simulink model "speed_ctrl"  (R2026a)
settings: Solver=ode4  StopTime=5  FixedStep=P_Ts/10
undefined symbols (not defined in the file or in its folder): P_alpha, P_cal, P_Dmax, P_dz, P_fm, P_Kb, P_Ki, P_Kp, P_omega_max, P_Rdn, P_Rup, P_Ts, PL_dz, PL_K, PL_Nrev, PL_tau, PL_td
settings Model: Creator=church  LastModifiedBy=church
settings DebuggingCC: ParameterPrecisionLossMsg=none

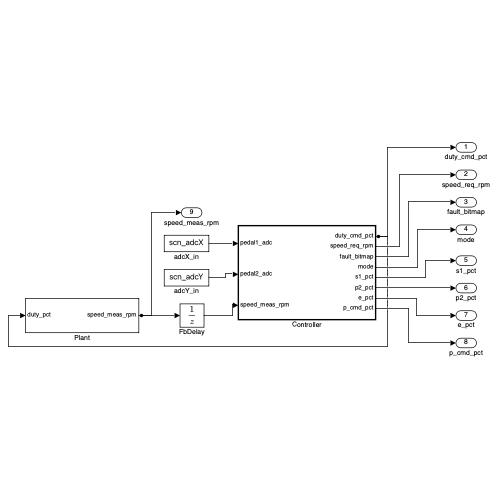
[thumbnail: Simulink's stored preview of the top-level diagram]
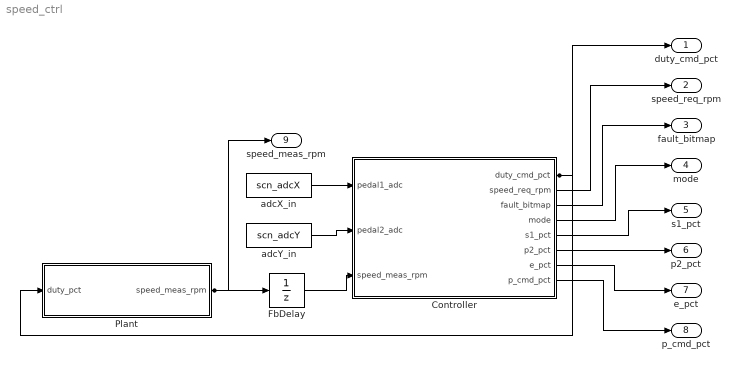
== system speed_ctrl ==
  Controller : Subsystem  TreatAsAtomicUnit=on
  FbDelay : UnitDelay  SampleTime=P_Ts
  Plant : Subsystem
  adcX_in : FromWorkspace  VariableName=scn_adcX  SampleTime=P_Ts  Interpolate=off  OutputAfterFinalValue=Holding final value
  adcY_in : FromWorkspace  VariableName=scn_adcY  SampleTime=P_Ts  Interpolate=off  OutputAfterFinalValue=Holding final value
  duty_cmd_pct : Outport  SampleTime=P_Ts
  speed_req_rpm : Outport  Port=2  SampleTime=P_Ts
  fault_bitmap : Outport  Port=3  SampleTime=P_Ts
  mode : Outport  Port=4  SampleTime=P_Ts
  s1_pct : Outport  Port=5  SampleTime=P_Ts
  p2_pct : Outport  Port=6  SampleTime=P_Ts
  e_pct : Outport  Port=7  SampleTime=P_Ts
  p_cmd_pct : Outport  Port=8  SampleTime=P_Ts
  speed_meas_rpm : Outport  Port=9  SampleTime=P_Ts
  wires:
  Controller/3(fault_bitmap) -> fault_bitmap/1
  Controller/5(s1_pct) -> s1_pct/1
  Controller/4(mode) -> mode/1
  Controller/6(p2_pct) -> p2_pct/1
  Controller/2(speed_req_rpm) -> speed_req_rpm/1
  Controller/7(e_pct) -> e_pct/1
  adcX_in/1 -> Controller/1(pedal1_adc)
  FbDelay/1 -> Controller/3(speed_meas_rpm)
  Plant/1(speed_meas_rpm) -> speed_meas_rpm/1, FbDelay/1
  Controller/8(p_cmd_pct) -> p_cmd_pct/1
  Controller/1(duty_cmd_pct) -> duty_cmd_pct/1, Plant/1(duty_pct)
  adcY_in/1 -> Controller/2(pedal2_adc)

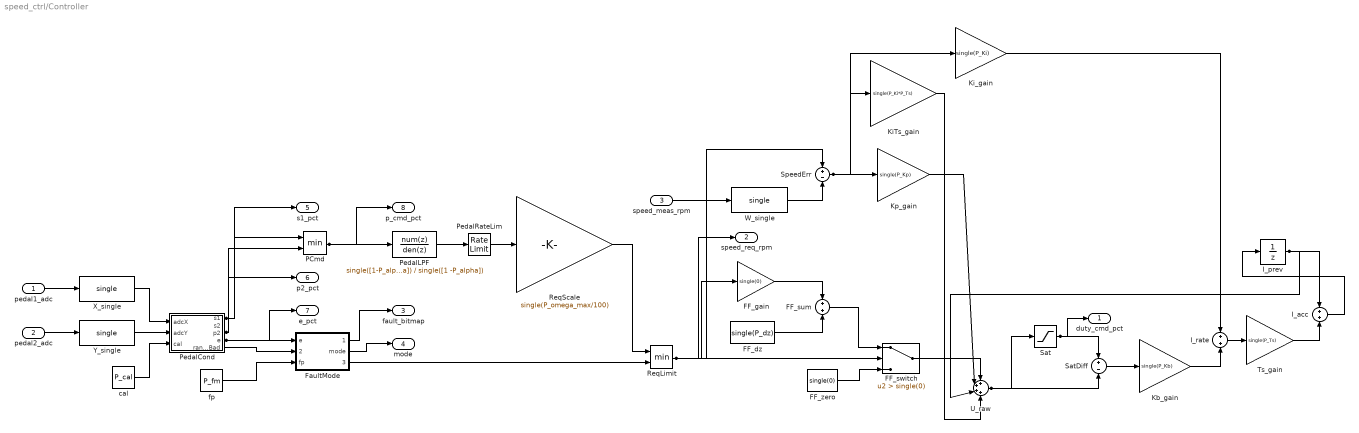
== system speed_ctrl/Controller ==
  pedal1_adc : Inport
  pedal2_adc : Inport  Port=2
  speed_meas_rpm : Inport  Port=3
  FF_dz : Constant  Value=single(P_dz)  OutDataTypeStr=single
  FF_gain : Gain  Gain=single(0)  ParamDataTypeStr=single
  FF_sum : Sum
  FF_switch : Switch  Criteria=u2 > Threshold  Threshold=single(0)  SaturateOnIntegerOverflow=off  InputSameDT=off
  FF_zero : Constant  Value=single(0)  OutDataTypeStr=single
  FaultMode : MATLAB Function  TreatAsAtomicUnit=on
  I_acc : Sum
  I_prev : UnitDelay  InitialCondition=single(0)  SampleTime=P_Ts
  I_rate : Sum
  Kb_gain : Gain  Gain=single(P_Kb)  ParamDataTypeStr=single
  KiTs_gain : Gain  Gain=single(P_Ki*P_Ts)  ParamDataTypeStr=single
  Ki_gain : Gain  Gain=single(P_Ki)  ParamDataTypeStr=single
  Kp_gain : Gain  Gain=single(P_Kp)  ParamDataTypeStr=single
  PCmd : MinMax  Inputs=2
  PedalCond : MATLAB Function  TreatAsAtomicUnit=on
  PedalLPF : DiscreteFilter  Numerator=single([1-P_alpha])  Denominator=single([1 -P_alpha])  SampleTime=P_Ts
  PedalRateLim : RateLimiter  RisingSlewLimit=single(P_Rup)  FallingSlewLimit=single(-P_Rdn)  SampleTimeMode=inherited
  ReqLimit : MinMax  Inputs=2
  ReqScale : Gain  Gain=single(P_omega_max/100)  ParamDataTypeStr=single
  Sat : Saturate  UpperLimit=single(P_Dmax)  LowerLimit=single(0)
  SatDiff : Sum  Inputs=+-
  SpeedErr : Sum  Inputs=+-
  Ts_gain : Gain  Gain=single(P_Ts)  ParamDataTypeStr=single
  U_raw : Sum  Inputs=++++
  W_single : DataTypeConversion  OutDataTypeStr=single  SaturateOnIntegerOverflow=off  RndMeth=Floor
  X_single : DataTypeConversion  OutDataTypeStr=single  SaturateOnIntegerOverflow=off  RndMeth=Floor
  Y_single : DataTypeConversion  OutDataTypeStr=single  SaturateOnIntegerOverflow=off  RndMeth=Floor
  cal : Constant  Value=P_cal  OutDataTypeStr=single
  fp : Constant  Value=P_fm  OutDataTypeStr=single
  duty_cmd_pct : Outport
  speed_req_rpm : Outport  Port=2
  fault_bitmap : Outport  Port=3
  mode : Outport  Port=4
  s1_pct : Outport  Port=5
  p2_pct : Outport  Port=6
  e_pct : Outport  Port=7
  p_cmd_pct : Outport  Port=8
  wires:
  I_rate/1 -> Ts_gain/1
  Kb_gain/1 -> I_rate/2
  SatDiff/1 -> Kb_gain/1
  Ki_gain/1 -> I_rate/1
  FF_switch/1 -> U_raw/1
  Kp_gain/1 -> U_raw/2
  KiTs_gain/1 -> U_raw/4
  FF_zero/1 -> FF_switch/3
  W_single/1 -> SpeedErr/2
  ReqLimit/1 -> speed_req_rpm/1, FF_switch/2, FF_gain/1, SpeedErr/1
  ReqScale/1 -> ReqLimit/1
  Ts_gain/1 -> I_acc/2
  speed_meas_rpm/1 -> W_single/1
  FaultMode/3(omega_lim) -> ReqLimit/2
  PedalRateLim/1 -> ReqScale/1
  FF_dz/1 -> FF_sum/2
  PedalLPF/1 -> PedalRateLim/1
  FaultMode/1(fault_bitmap) -> fault_bitmap/1
  PedalCond/5(rangeBad) -> FaultMode/2(rangeBad)
  pedal2_adc/1 -> Y_single/1
  PedalCond/3(p2) -> p2_pct/1, PCmd/2
  Sat/1 -> duty_cmd_pct/1, SatDiff/1
  PedalCond/1(s1) -> s1_pct/1, PCmd/1
  X_single/1 -> PedalCond/1(adcX)
  I_prev/1 -> I_acc/1, U_raw/3
  PedalCond/4(e) -> e_pct/1, FaultMode/1(e)
  I_acc/1 -> I_prev/1
  U_raw/1 -> Sat/1, SatDiff/2
  FF_gain/1 -> FF_sum/1
  cal/1 -> PedalCond/3(cal)
  SpeedErr/1 -> KiTs_gain/1, Kp_gain/1, Ki_gain/1
  fp/1 -> FaultMode/3(fp)
  FF_sum/1 -> FF_switch/1
  Y_single/1 -> PedalCond/2(adcY)
  FaultMode/2(mode) -> mode/1
  PCmd/1 -> p_cmd_pct/1, PedalLPF/1
  pedal1_adc/1 -> X_single/1

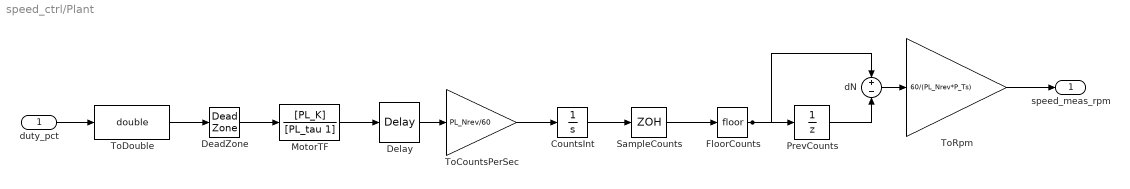
== system speed_ctrl/Plant ==
  duty_pct : Inport
  CountsInt : Integrator
  DeadZone : DeadZone  LowerValue=-PL_dz  UpperValue=PL_dz
  Delay : TransportDelay  DelayTime=PL_td
  FloorCounts : Rounding
  MotorTF : TransferFcn  Numerator=[PL_K]  Denominator=[PL_tau 1]
  PrevCounts : UnitDelay  SampleTime=P_Ts
  SampleCounts : ZeroOrderHold  SampleTime=P_Ts
  ToCountsPerSec : Gain  Gain=PL_Nrev/60
  ToDouble : DataTypeConversion  OutDataTypeStr=double  SaturateOnIntegerOverflow=off  RndMeth=Floor
  ToRpm : Gain  Gain=60/(PL_Nrev*P_Ts)
  dN : Sum  Inputs=+-
  speed_meas_rpm : Outport
  wires:
  ToRpm/1 -> speed_meas_rpm/1
  dN/1 -> ToRpm/1
  SampleCounts/1 -> FloorCounts/1
  duty_pct/1 -> ToDouble/1
  PrevCounts/1 -> dN/2
  CountsInt/1 -> SampleCounts/1
  ToCountsPerSec/1 -> CountsInt/1
  FloorCounts/1 -> PrevCounts/1, dN/1
  ToDouble/1 -> DeadZone/1
  Delay/1 -> ToCountsPerSec/1
  DeadZone/1 -> MotorTF/1
  MotorTF/1 -> Delay/1

== matlab function speed_ctrl/Controller/FaultMode ==
  data: e input; fault_bitmap output; rangeBad input; fp input; mode output; omega_lim output
function [fault_bitmap, mode, omega_lim] = FaultMode(e, rangeBad, fp)
% fp = [Dpl Npl Nrange Nclear omega_max omega_limp]
persistent cPl aPl cRg aRg cClr modeS
if isempty(cPl)
    cPl = single(0); aPl = false; cRg = single(0); aRg = false; cClr = single(0); modeS = uint8(0);
end
if e > fp(1), cPl = min(cPl + single(1), fp(2)); else, cPl = max(cPl - single(1), single(0)); end
if cPl >= fp(2), aPl = true; end
if cPl <= single(0), aPl = false; end
if rangeBad, cRg = min(cRg + single(1), fp(3)); else, cRg = max(cRg - single(1), single(0)); end
if cRg >= fp(3), aRg = true; end
if cRg <= single(0), aRg = false; end
if aPl || aRg
    cClr = single(0); modeS = uint8(1);
elseif modeS == uint8(1)
    cClr = cClr + single(1);
    if cClr >= fp(4), modeS = uint8(0); end
end
fault_bitmap = uint16(0);
if aPl, fault_bitmap = bitor(fault_bitmap, uint16(1)); end
if aRg, fault_bitmap = bitor(fault_bitmap, uint16(2)); end
mode = modeS;
if modeS == uint8(0), omega_lim = fp(5); else, omega_lim = fp(6); end

== matlab function speed_ctrl/Controller/PedalCond ==
  data: adcX input; s1 output; adcY input; cal input; s2 output; p2 output; e output; rangeBad output
function [s1,s2,p2,e,rangeBad] = PedalCond(adcX, adcY, cal)
[s1,s2,p2,e,rangeBad] = pedal_cond_core(adcX, adcY, cal);
